simulink model "sfInternalTransitionFixed"  (R2025b)
settings: Solver=VariableStepAuto  StartTime=0.0  StopTime=10.0  RelTol=1e-3
settings Model: Creator=The MathWorks, Inc.  LastModifiedBy=The MathWorks, Inc.

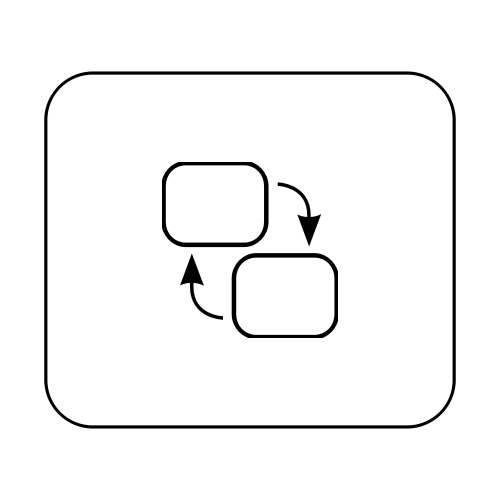
[thumbnail: Simulink's stored preview of the top-level diagram]
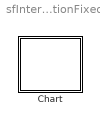
== system sfInternalTransitionFixed ==
  Chart : Stateflow chart  TreatAsAtomicUnit=on

== stateflow chart sfInternalTransitionFixed/Chart ==
  state B [parallel]
    settings: executionOrder=1
    state A
    (default) -> A
    A -> (junction 15) : every(1,tick)
    (junction 16) -> A : {x=x+3;}
    (junction 15) -> (junction 16)
  state C [parallel]
    settings: executionOrder=2
    C -> (junction 23) : every(1,tick){x=x+1; send(local,B);}
  data: x local =0
  events: local local FUNCTION_CALL_EVENT
